simulink model "backup222"  (R2025a)
settings: Solver=ode4  StartTime=0.0  StopTime=10  FixedStep=0.0005  RelTol=1e-3
InitFcn:
  | Electronic_stability_program_model_parameter;
undefined symbols (not defined in the file): A, B, canChannel
libraries: canlib x5, canmsglib x4, Solver_SF x1, sldrtlib x1, simulink x1
settings Model: SimulationMode=external  Creator=LXR  LastModifiedBy=65365
settings SolverCC: AlgebraicLoopSolver=TrustRegion
settings HardwareCC: ProdBitPerLong=64.0  ProdHWDeviceType=Intel->x86-64 (Linux 64)
settings RTWCC: SystemTargetFile=sldrt.tlc  TemplateMakefile=sldrt.tmf  RTWCompilerOptimization=on  GPUComputeCapability=3.5  Description=Simulink Desktop Real-Time
settings CodeAppCC: MaxIdLength=95.0
settings SimulinkDesktopRealTimeCC: ExtModeTransport=0.0  ExtModeStaticAllocSize=1000000.0  TargetLibSuffix=_sldrt.a  TargetPreCompLibLocation=F:\toolbox\sldrt\lib\win64  MultiwordLength=2048.0  DynamicStringBufferSize=256.0  ParMdlRefBuildCompliant=on  PreserveMATLABNamespacesInGeneratedCode=on  SubcomponentCodeInterfacePackaging=Reusable function

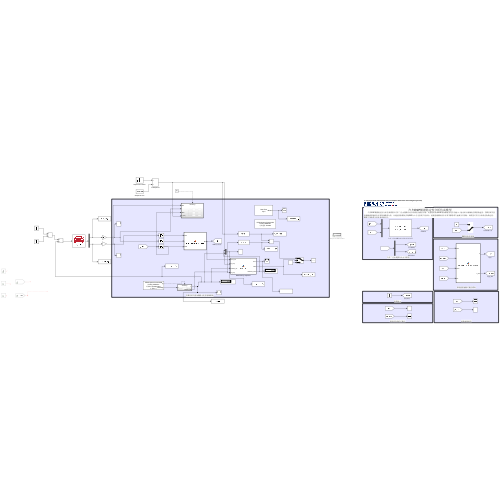
[thumbnail: Simulink's stored preview of the top-level diagram]
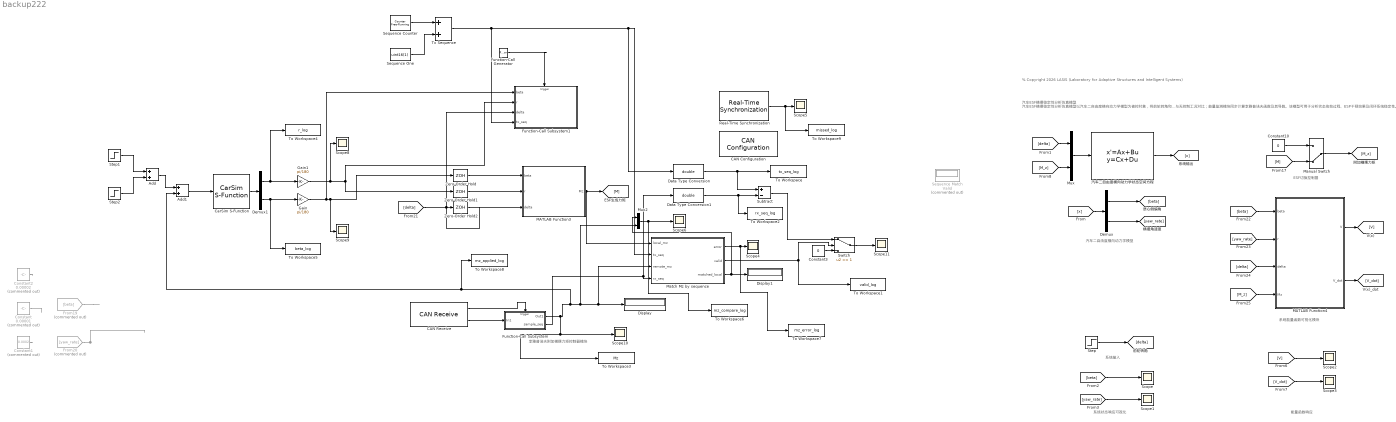
== system backup222 ==
  note: 李雅普诺夫附加横摆力矩控制器模块
  note: ESP切换控制器
  note: 能量函数响应
  note: 系统能量函数可视化模块
  note: 汽车二自由度横向动力学模型
  note: 系统输入
  note: 系统状态响应可视化
  note: 汽车ESP横摆稳定性分析仿真模型
      | 汽车ESP横摆稳定性分析仿真模型以汽车二自由度横向动力学模型为被控对象，将前轮转角和ESP附加横摆力矩作为输入，输出质心侧偏角与横摆角速度。李雅普诺夫控制器根据车辆状态计算附加横摆力矩，并通过切换模块实现ESP介入与无控制工况对比；能量监测模块同步计算李雅普诺夫函数及其导数。该模型可用于分析状态收敛过程、ESP干预效果及闭环系统稳定性。
  note: % Copyright 2026 LASIS (Laboratory for Adaptive Structures and Intelligent Systems)
  Add : Sum
  Add1 : Sum
  CAN Configuration : canlib/CAN Configuration  BlockHandle=285.0001  Device=PEAK-System PCAN-USB (PCAN_USBBUS1)  DeviceMenu=PEAK-System PCAN-USB (PCAN_USBBUS1)  ObjConstructor=canChannel('PEAK-System', 'PCAN_USBBUS1')  BusSpeed=500000  EnableBitParameters=off  AckMode=Normal
  CAN Receive : canlib/CAN Receive  BlockHandle=286.0001  Device=PEAK-System PCAN-USB (PCAN_USBBUS1)  DeviceMenu=PEAK-System PCAN-USB (PCAN_USBBUS1)  ObjConstructor=canChannel('PEAK-System', 'PCAN_USBBUS1')  EnableStandardIDsFilter=off  StdIDsCombo=Allow only  StandardIDs=hex2dec('203')  EnableExtendedIDsFilter=off  ExtIDsCombo=Block all  ExtendedIDs=0  SampleTime=0.0005  MsgsPerTimestep=all  InternalFilterUpdateStatus=on  BusOutput=off
  CarSim S-Function : Solver_SF/CarSim S-Function  Priority=1  SIMFILE=simfile.sim  Run_RTs=off  vs_state_ind=Run  StopMode_ind=Vehicle Model
  Constant : Constant  Commented=on  Value=0.00001  SampleTime=0.01
  Constant1 : Constant  Commented=on  Value=0.0002  SampleTime=0.01
  Constant10 : Constant  Value=0
  Constant2 : Constant  Commented=on  Value=0.00002  SampleTime=0.01
  Constant3 : Constant  Value=0
  Data Type Conversion : DataTypeConversion  OutDataTypeStr=double  SaturateOnIntegerOverflow=off  RndMeth=Floor
  Data Type Conversion1 : DataTypeConversion  OutDataTypeStr=double  SaturateOnIntegerOverflow=off  RndMeth=Floor
  Demux : Demux  Outputs=2
  Demux1 : Demux  Outputs=2
  Display : Display
  Display1 : Display
  From19 : From  Commented=on  GotoTag=beta
  From20 : From  Commented=on  GotoTag=yaw_rate
  Function-Call Generator : FunctionCallGenerator  SampleTime=0.01
  Function-Call Subsystem : Subsystem  TreatAsAtomicUnit=on
  Function-Call Subsystem1 : Subsystem  TreatAsAtomicUnit=on
  Gain : Gain  Gain=pi/180
  Gain1 : Gain  Gain=pi/180
  MATLAB Function3 : MATLAB Function  TreatAsAtomicUnit=on
  MATLAB Function4 : MATLAB Function  TreatAsAtomicUnit=on
  Manual Switch : ManualSwitch  CurrentSetting=0
  Match Mz by sequence : MATLAB Function  TreatAsAtomicUnit=on
  Mux : Mux  Inputs=2
  Mux2 : Mux  Inputs=2
  Real-Time Synchronization : sldrtlib/Real-Time Synchronization  SampleTime=0.01  MaxMissedTicks=100  ShowMissedTicks=on  YieldWhenWaiting=off
  Scope{,1..6,8..11} (11 alike) : Scope
      Scope settings: ActiveDisplayYMinimum=-0.012500538434860898  ActiveDisplayYMaximum=0.11250005982609566
      Scope1 settings: ActiveDisplayYMinimum=-0.029279023350753913  ActiveDisplayYMaximum=0.5761499870872272
      Scope10 settings: ActiveDisplayYMinimum=-4693.2955322265625  ActiveDisplayYMaximum=2239.6597900390625  DataLoggingVariableName=ScopeData10
      Scope11 settings: ActiveDisplayYMinimum=-0.62499999999999989  ActiveDisplayYMaximum=5.625  DataLoggingVariableName=ScopeData11
      Scope2 settings: ActiveDisplayYMinimum=-150.7307  ActiveDisplayYMaximum=1433.4145  DataLoggingVariableName=ScopeData2
      Scope3 settings: ActiveDisplayYMinimum=-11697.2812  ActiveDisplayYMaximum=1299.6942  DataLoggingVariableName=ScopeData3
      Scope4 settings: ActiveDisplayYMinimum=-5.0746523555744716E-5  ActiveDisplayYMaximum=9.0419989163592618E-5  DataLoggingVariableName=ScopeData4
      Scope5 settings: ActiveDisplayYMinimum=-2.7499999999999996  ActiveDisplayYMaximum=24.75  DataLoggingVariableName=ScopeData5
      Scope6 settings: ActiveDisplayYMinimum=-1279.8107833862305  ActiveDisplayYMaximum=907.60124969482422  DataLoggingVariableName=ScopeData6
      Scope8 settings: ActiveDisplayYMinimum=-0.0070389833953762122  ActiveDisplayYMaximum=0.0367533080502689  DataLoggingVariableName=ScopeData8
      Scope9 settings: ActiveDisplayYMinimum=-0.00034776827620076461  ActiveDisplayYMaximum=4.0304969255946E-5  DataLoggingVariableName=ScopeData9
  Sequence Counter : simulink/Sources/Counter Free-Running  NumBits=16  tsamp=0.01
  Sequence Match Valid : Display  Commented=on
  Sequence One : Constant  Value=uint16(1)  OutDataTypeStr=uint16
  Step : Step  After=0  SampleTime=0
  Step1 : Step  After=1000  SampleTime=0
  Step2 : Step  Time=1.1  After=-1000  SampleTime=0
  Subtract : Sum  Inputs=+-
  Switch : Switch  Threshold=1  SaturateOnIntegerOverflow=off  InputSameDT=off
  To Workspace : ToWorkspace  VariableName=tx_seq_log  SaveFormat=Timeseries  SampleTime=-1
  To Workspace1 : ToWorkspace  VariableName=valid_log  SaveFormat=Timeseries  SampleTime=-1
  To Workspace2 : ToWorkspace  VariableName=rx_seq_log  SaveFormat=Timeseries  SampleTime=-1
  To Workspace3 : ToWorkspace  VariableName=Mz  SaveFormat=Timeseries  SampleTime=-1
  To Workspace4 : ToWorkspace  VariableName=r_log  SaveFormat=Timeseries  SampleTime=-1
  To Workspace5 : ToWorkspace  VariableName=beta_log  SaveFormat=Timeseries  SampleTime=-1
  To Workspace6 : ToWorkspace  VariableName=mz_compare_log  SaveFormat=Timeseries  SampleTime=-1
  To Workspace7 : ToWorkspace  VariableName=mz_error_log  SaveFormat=Timeseries  SampleTime=-1
  To Workspace8 : ToWorkspace  VariableName=mz_applied_log  SaveFormat=Timeseries  SampleTime=-1
  To Workspace9 : ToWorkspace  VariableName=missed_log  SaveFormat=Timeseries  SampleTime=-1
  Tx Sequence : Sum  OutDataTypeStr=uint16
  Zero-Order Hold : ZeroOrderHold  SampleTime=0.01
  Zero-Order Hold1 : ZeroOrderHold  SampleTime=0.01
  Zero-Order Hold2 : ZeroOrderHold  SampleTime=0.01
  汽车二自由度横向动力学状态空间方程 : StateSpace  A=A  B=B  C=eye(2)  D=[0,0;0,0]  InitialCondition=[0.1;0.5]
  wires:
  Demux/2 -> [yaw_rate]
  Demux/1 -> [beta]
  Step/1 -> [delta]
  [beta] -> Scope/1
  [yaw_rate] -> Scope1/1
  [x] -> Demux/1
  [V] -> Scope2/1
  [V_dot] -> Scope3/1
  Mux/1 -> 汽车二自由度横向动力学状态空间方程/1
  汽车二自由度横向动力学状态空间方程/1 -> [x]
  Constant10/1 -> Manual Switch/1
  [delta] -> Mux/1
  [M_z] -> Mux/2
  Manual Switch/1 -> [M_z]
  [M] -> Manual Switch/2
  MATLAB Function3/1(Mz) -> [M], Match Mz by sequence/1(local_mz)
  [beta] -> MATLAB Function4/1(beta)
  [yaw_rate] -> MATLAB Function4/2(r)
  [delta] -> MATLAB Function4/3(delta)
  [M_z] -> MATLAB Function4/4(Mz)
  MATLAB Function4/1(V) -> [V]
  MATLAB Function4/2(V_dot) -> [V_dot]
  Real-Time Synchronization/1 -> To Workspace9/1, Scope5/1
  From19/1 -> ?
  Zero-Order Hold/1 -> MATLAB Function3/1(beta)
  From20/1 -> ?
  [delta] -> Zero-Order Hold2/1
  Zero-Order Hold1/1 -> MATLAB Function3/2(r)
  Zero-Order Hold2/1 -> Function-Call Subsystem1/3(delta), MATLAB Function3/3(delta)
  Constant/1 -> ?
  Constant1/1 -> ?
  Constant2/1 -> ?
  CAN Receive/1 -> Function-Call Subsystem/Trigger
  CAN Receive/2 -> Function-Call Subsystem/1(In1)
  Function-Call Subsystem/1(Out1) -> To Workspace3/1, Scope10/1, Add1/2, To Workspace8/1, Mux2/2, Match Mz by sequence/3(remote_mz), Display/1
  Function-Call Subsystem/2(sample_seq) -> Data Type Conversion1/1, Match Mz by sequence/4(rx_seq)
  Match Mz by sequence/1(error) -> To Workspace7/1, Scope4/1
  Match Mz by sequence/2(valid) -> Switch/2, To Workspace1/1
  Mux2/1 -> Scope6/1, To Workspace6/1
  Match Mz by sequence/3(matched_local) -> Mux2/1, Display1/1
  CarSim S-Function/1 -> Demux1/1
  Demux1/1 -> To Workspace4/1, Gain1/1
  Demux1/2 -> Gain/1, To Workspace5/1
  Step2/1 -> Add/2
  Step1/1 -> Add/1
  Add/1 -> Add1/1
  Add1/1 -> CarSim S-Function/1
  Gain1/1 -> Function-Call Subsystem1/2(r), Zero-Order Hold1/1, Scope8/1
  Gain/1 -> Function-Call Subsystem1/1(beta), Zero-Order Hold/1, Scope9/1
  Data Type Conversion/1 -> To Workspace/1, Subtract/1
  Data Type Conversion1/1 -> To Workspace2/1, Subtract/2
  Subtract/1 -> Switch/1
  Switch/1 -> Scope11/1
  Constant3/1 -> Switch/3
  Function-Call Generator/1 -> Function-Call Subsystem1/Trigger
  Sequence Counter/1 -> Tx Sequence/1
  Sequence One/1 -> Tx Sequence/2
  Tx Sequence/1 -> Data Type Conversion/1, Match Mz by sequence/2(tx_seq), Function-Call Subsystem1/4(tx_seq)

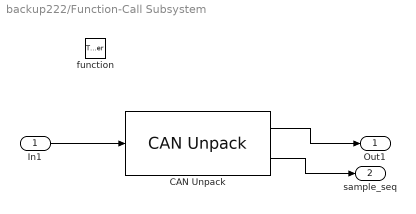
== system backup222/Function-Call Subsystem ==
  In1 : Inport
  function : TriggerPort  TriggerType=function-call  VariantControl=(inherit)
  CAN Unpack : canmsglib/CAN Unpack  CANdbFile=D:\Lab\step1\vehicle_controller.dbc  MsgList=Controller_Output  MsgName=Controller_Output  MsgIDType=Standard (11-bit identifier)  MsgIdentifier=515  MsgLength=6  SignalInfo="{ 'M', '0', '32', 'LE', 'single', 'Standard', '0', '1', '0', '-Inf', 'Inf';          'sample_seq', '32', '16', 'LE', 'unsigned', 'Standard', '0', '1', '0', '0', '65535' }"  IDPort=off  TimestampPort=off  ErrorPort=off  RemotePort=off  LengthPort=off  StatusPort=off  ApplyMinMax=off
      settings: LibrarySourceBlock=canlib/CAN Unpack
  Out1 : Outport
  sample_seq : Outport  Port=2
  wires:
  In1/1 -> CAN Unpack/1
  CAN Unpack/1 -> Out1/1
  CAN Unpack/2 -> sample_seq/1

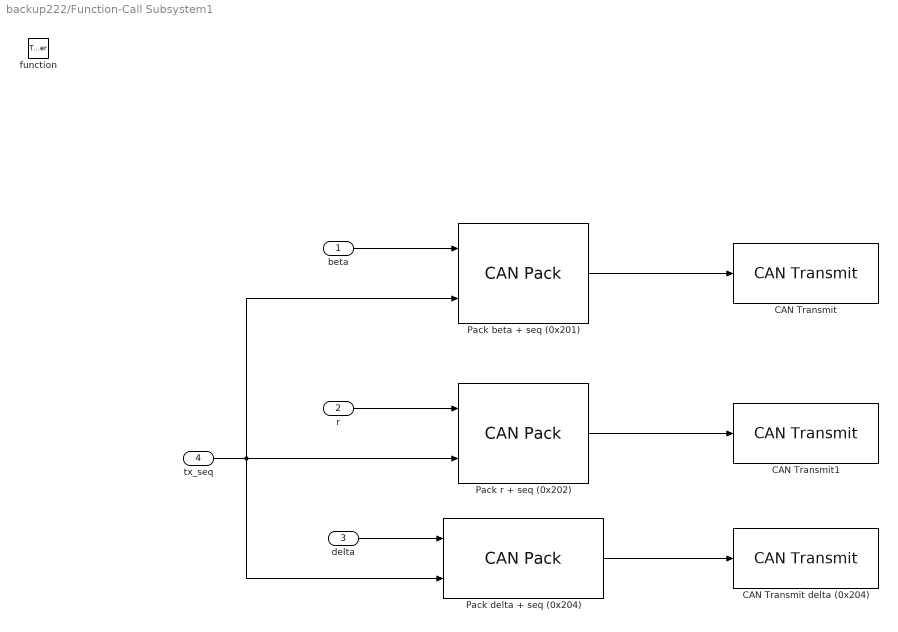
== system backup222/Function-Call Subsystem1 ==
  beta : Inport
  r : Inport  Port=2
  delta : Inport  Port=3
  tx_seq : Inport  Port=4
  function : TriggerPort  TriggerType=function-call  VariantControl=(inherit)
  CAN Transmit : canlib/CAN Transmit  Priority=1  BlockHandle=388.0001  Device=PEAK-System PCAN-USB (PCAN_USBBUS1)  DeviceMenu=PEAK-System PCAN-USB (PCAN_USBBUS1)  ObjConstructor=canChannel('PEAK-System', 'PCAN_USBBUS1')  EnableEventTransmit=off  EnablePeriodicTransmit=off  MessagePeriod=0.01
  CAN Transmit delta (0x204) : canlib/CAN Transmit  Priority=3  BlockHandle=390.0001  Device=PEAK-System PCAN-USB (PCAN_USBBUS1)  DeviceMenu=PEAK-System PCAN-USB (PCAN_USBBUS1)  ObjConstructor=canChannel('PEAK-System', 'PCAN_USBBUS1')  EnableEventTransmit=off  EnablePeriodicTransmit=off  MessagePeriod=0.01
  CAN Transmit1 : canlib/CAN Transmit  Priority=2  BlockHandle=392.0001  Device=PEAK-System PCAN-USB (PCAN_USBBUS1)  DeviceMenu=PEAK-System PCAN-USB (PCAN_USBBUS1)  ObjConstructor=canChannel('PEAK-System', 'PCAN_USBBUS1')  EnableEventTransmit=off  EnablePeriodicTransmit=off  MessagePeriod=0.01
  Pack beta + seq (0x201) : canmsglib/CAN Pack  CANdbFile=D:\Lab\step1\vehicle_controller.dbc  MsgList=Controller_Input  MsgName=Controller_Input  MsgIDType=Standard (11-bit identifier)  MsgIdentifier=513  CANIDInput=off  MsgLength=6  Remote=off  ApplyMinMax=off  BusOutput=off  SignalInfo="{ 'beta', '0', '32', 'LE', 'single', 'Standard', '0', '1', '0', '-Inf', 'Inf';     'seq_beta', '32', '16', 'LE', 'unsigned', 'Standard', '0', '1', '0', '0', '65535' }"
      settings: LibrarySourceBlock=canlib/CAN Pack  DataFormat=manually specified signals
  Pack delta + seq (0x204) : canmsglib/CAN Pack  CANdbFile=D:\Lab\step1\vehicle_controller.dbc  MsgList=Controller_Input  MsgName=Controller_Input  MsgIDType=Standard (11-bit identifier)  MsgIdentifier=516  CANIDInput=off  MsgLength=6  Remote=off  ApplyMinMax=off  BusOutput=off  SignalInfo="{ 'delta', '0', '32', 'LE', 'single', 'Standard', '0', '1', '0', '-Inf', 'Inf';     'seq_delta', '32', '16', 'LE', 'unsigned', 'Standard', '0', '1', '0', '0', '65535' }"
      settings: LibrarySourceBlock=canlib/CAN Pack  DataFormat=manually specified signals
  Pack r + seq (0x202) : canmsglib/CAN Pack  CANdbFile=D:\Lab\step1\vehicle_controller.dbc  MsgList=Controller_Input  MsgName=Controller_Input_Delta  MsgIDType=Standard (11-bit identifier)  MsgIdentifier=514  CANIDInput=off  MsgLength=6  Remote=off  ApplyMinMax=off  BusOutput=off  SignalInfo={ 'yaw_rate', '0', '32', 'LE', 'single', 'Standard', '0', '1', '0', '-Inf', 'Inf'; 'seq_r', '32', '16', 'LE', 'unsigned', 'Standard', '0', '1', '0', '0', '65535' }
      settings: LibrarySourceBlock=canlib/CAN Pack  DataFormat=manually specified signals
  wires:
  Pack beta + seq (0x201)/1 -> CAN Transmit/1
  beta/1 -> Pack beta + seq (0x201)/1
  Pack r + seq (0x202)/1 -> CAN Transmit1/1
  r/1 -> Pack r + seq (0x202)/1
  Pack delta + seq (0x204)/1 -> CAN Transmit delta (0x204)/1
  delta/1 -> Pack delta + seq (0x204)/1
  tx_seq/1 -> Pack beta + seq (0x201)/2, Pack delta + seq (0x204)/2, Pack r + seq (0x202)/2

== matlab function backup222/Match Mz by sequence ==
  data: local_mz input; error output; tx_seq input; remote_mz input; rx_seq input; valid output; matched_local output
function [error, valid, matched_local] = match_mz(local_mz, tx_seq, remote_mz, rx_seq)
%#codegen
persistent mz_cache seq_cache slot_valid
if isempty(mz_cache)
    mz_cache = zeros(256,1);
    seq_cache = zeros(256,1,'uint16');
    slot_valid = false(256,1);
end
tx_idx = double(bitand(uint16(tx_seq),uint16(255))) + 1;
mz_cache(tx_idx) = double(local_mz);
seq_cache(tx_idx) = uint16(tx_seq);
slot_valid(tx_idx) = true;
rx_idx = double(bitand(uint16(rx_seq),uint16(255))) + 1;
if slot_valid(rx_idx) && seq_cache(rx_idx) == uint16(rx_seq) && uint16(rx_seq) ~= uint16(0)
    matched_local = mz_cache(rx_idx);
    error = matched_local - double(remote_mz);
    valid = true;
else
    matched_local = 0;
    error = 0;
    valid = false;
end

== matlab function backup222/MATLAB Function3 ==
  data: beta input; r input; delta input; Mz output
function Mz = direct_lyapunov_controller(beta, r, delta)
    % 1. 车辆参数定义 
    m = 1750; Iz = 3000; a = 1.25; b = 1.45;
    kf = 65000; kr = 45000; vx = 30;
    
    % 2. 设定期望的能量耗散速度 (可调参数)
    K1 = 500000;         % 对应 beta 的衰减力度
    K2 = 500000;         % 对应 r 的衰减力度
    epsilon = 0.00001;    % 极小保护阈值
    % 3. 实时计算当前轮胎侧向力
    Fyf = kf * (delta - beta - a * r / vx);
    Fyr = kr * (-beta + b * r / vx);

    if abs(r) < epsilon
        if r >= 0
            r_safe = epsilon;
        else
            r_safe = -epsilon;
        end
    else
        r_safe = r;
    end
    
    % 4. 严格执行李雅普诺夫代数解公式
    term1 = -K1 * beta^2 - K2 * r_safe^2;
    term2 = -2 * beta * (Fyf + Fyr - m * vx * r_safe);
    
    Mz_raw = (term1 + term2) /(2 * r_safe )  - (a * Fyf - b * Fyr);
    
    % 5. 物理限幅 
    if Mz_raw > 4000
        Mz = 4000;
    elseif Mz_raw < -4000
        Mz = -4000;
    else
        Mz = Mz_raw;
    end
end

== matlab function backup222/MATLAB Function4 ==
  data: beta input; V output; r input; delta input; Mz input; V_dot output
function [V, V_dot] = Analytical_Lyapunov_Observer(beta, r, delta, Mz)
    % 1. 统一的车辆参数 
    m = 1750; Iz = 3000; a = 1.25; b = 1.45; vx = 30;
    kf = 65000; kr = 45000; mu = 0.8; g = 9.8;
    
    % 2. 内部重构轮胎受力
    Fzf = m * g * b / (a + b);
    Fzr = m * g * a / (a + b);
    Fmax_f = mu * Fzf;
    Fmax_r = mu * Fzr;
    
    alpha_f = delta - beta - a * r / vx;
    alpha_r = -beta + b * r / vx;
    
    Fyf = Fmax_f * tanh(kf * alpha_f / Fmax_f);
    Fyr = Fmax_r * tanh(kr * alpha_r / Fmax_r);
    
    % 3. 利用动力学解析方程计算导数
    beta_dot = (Fyf + Fyr) / (m * vx) - r;
    r_dot = (a * Fyf - b * Fyr + Mz) / Iz;
    
    % 4. 计算并输出李雅普诺夫函数值及导数值
    V = m * vx * beta^2 + Iz * r^2;
    V_dot = 2 * m * vx * beta * beta_dot + 2 * Iz * r * r_dot;
    
end
